simulink model "TP8_gestion_allumage_moteur"  (R2022b)
settings: Solver=VariableStepAuto  StartTime=0.0  StopTime=25  RelTol=1e-3
libraries: simulink x8, fl_lib x7, nesl_utility x4, ee_lib x2
settings Model: Creator=HP  LastModifiedBy=HP

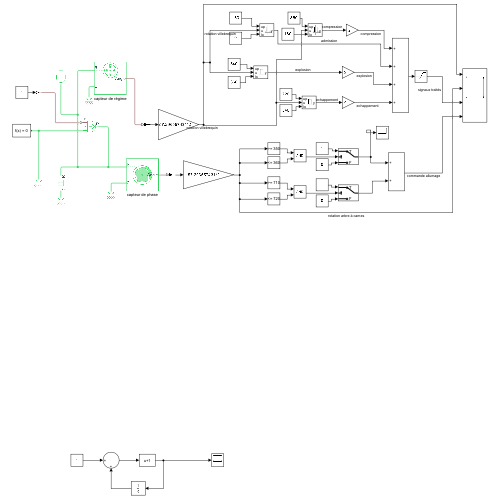
[thumbnail: Simulink's stored preview of the top-level diagram]
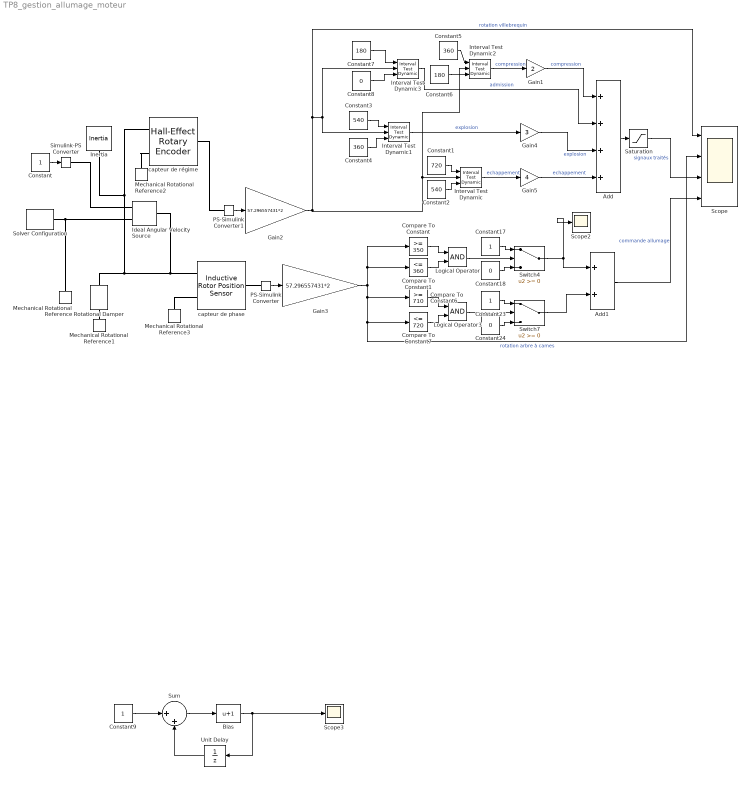
== system TP8_gestion_allumage_moteur ==
  Add : Sum  Inputs=++++
  Add1 : Sum
  Bias : Bias  Bias=1  SaturateOnIntegerOverflow=off
  Compare To Constant : simulink/Logic and Bit Operations/Compare To Constant  relop=>=  const=350  OutDataTypeStr=boolean
  Compare To Constant1 : simulink/Logic and Bit Operations/Compare To Constant  relop=<=  const=360  OutDataTypeStr=boolean
  Compare To Constant6 : simulink/Logic and Bit Operations/Compare To Constant  relop=>=  const=710  OutDataTypeStr=boolean
  Compare To Constant7 : simulink/Logic and Bit Operations/Compare To Constant  relop=<=  const=720  OutDataTypeStr=boolean
  Constant{,9,17,23} (4 alike) : Constant
  Constant1 : Constant  Value=720
  Constant18 : Constant  Value=0
  Constant2 : Constant  Value=540
  Constant24 : Constant  Value=0
  Constant3 : Constant  Value=540
  Constant4 : Constant  Value=360
  Constant5 : Constant  Value=360
  Constant6 : Constant  Value=180
  Constant7 : Constant  Value=180
  Constant8 : Constant  Value=0
  Gain1 : Gain  Gain=2
  Gain2 : Gain  Gain=57.296557431*2
  Gain3 : Gain  Gain=57.296557431*2
  Gain4 : Gain  Gain=3
  Gain5 : Gain  Gain=4
  Ideal Angular Velocity Source : fl_lib/Mechanical/Mechanical Sources/Ideal Angular Velocity Source
  Inertia : fl_lib/Mechanical/Rotational Elements/Inertia  inertia=0.01 kg*m^2  num_ports=foundation.enum.numPorts2.one  w_specify=on  w_priority=None  w=0 rad/s  w_nominal_specify=off  w_nominal_unit=rad/s  w_nominal_value=1  t_specify=off  t_priority=None  t=0 N*m  t_nominal_specify=off  t_nominal_unit=N*m  t_nominal_value=1
  Interval Test Dynamic{,1..3} (4 alike) : simulink/Logic and Bit Operations/Interval Test Dynamic  IntervalClosedRight=on  IntervalClosedLeft=on  OutDataTypeStr=boolean
  Logical Operator : Logic  AllPortsSameDT=off  OutDataTypeStr=boolean
  Logical Operator3 : Logic  AllPortsSameDT=off  OutDataTypeStr=boolean
  Mechanical Rotational Reference{,1..3} (4 alike) : fl_lib/Mechanical/Rotational Elements/Mechanical Rotational Reference
  PS-Simulink Converter : nesl_utility/PS-Simulink Converter  PhysicalDomain=network_engine_domain  SubClassName=ps_output  LeftPortType=input  RightPortType=output  PseudoPeriodic=off  Frequencies=[]  VectorFormat=inherit  Unit=inherit  AffineConversion=off
  PS-Simulink Converter1 : nesl_utility/PS-Simulink Converter  PhysicalDomain=network_engine_domain  SubClassName=ps_output  LeftPortType=input  RightPortType=output  PseudoPeriodic=off  Frequencies=[]  VectorFormat=inherit  Unit=inherit  AffineConversion=off
  Rotational Damper : fl_lib/Mechanical/Rotational Elements/Rotational Damper  D=0.001 N*m*s/rad  w_specify=off  w_priority=None  w=0 rad/s  w_nominal_specify=off  w_nominal_unit=rad/s  w_nominal_value=1  t_specify=off  t_priority=None  t=0 N*m  t_nominal_specify=off  t_nominal_unit=N*m  t_nominal_value=1
  Saturation : Saturate  UpperLimit=4  LowerLimit=1
  Scope : Scope  NumInputPorts=4
  Scope2 : Scope
  Scope3 : Scope
  Simulink-PS Converter : nesl_utility/Simulink-PS Converter  PhysicalDomain=network_engine_domain  SubClassName=ps_input  LeftPortType=input  RightPortType=output  PseudoPeriodic=off  Frequencies=[]  NoiseDistribution=none  NoiseParameters=[]  Unit=1  AffineConversion=off  FilteringAndDerivatives=provide  SimscapeFilterOrder=1  InputFilterTimeConstant=0.001  UdotUserProvided=0
  Solver Configuration : nesl_utility/Solver Configuration  PhysicalDomain=network_engine_domain  SubClassName=solver  LeftPortType=input  RightPortType=generic  Tones=[]  Harmonics=[]  SimulateNoise=off  Profile=off  UseLocalSampling=off  EnableSwitchedLinearOptims=on  FrequencyDomain=off  UseCCode=off  RelTol=0.001  AbsTol=0.001  MinStep=1e-09  ToWorkspace=off  RevertToSquareIcSolve=off  NumHomotopyIterations=100  PhasorMode=off  PhasorModeNumHarmonics=1  ConsistencySolver=NEWTON_XTOL_AFTER_FTOL  IndexReductionMethod=DerivativeReplacement  DoDC=off  ResidualTolerance=1e-09  ConsistencyTolSource=GLOBAL  ConsistencyAbsTol=0.001  ConsistencyRelTol=0.001  ConsistencyTolFactor=0.001  UseLocalSolver=off  LocalSolverChoice=NE_BACKWARD_EULER_ADVANCER  ResolveIndetEquations=on  FunctionEvalNumThread=1  LocalSolverSampleTime=0.001  DoFixedCost=off  MaxNonlinIter=3  MaxModeIter=2  ComputeImpulses=off  ImpulseIterations=2  LinearAlgebra=auto  LinearAlgebraNumThread=0  EquationFormulation=NE_TIME_EF  DelaysMemoryBudget=1024  AutomaticFiltering=on  FilteringTimeConstant=0.001  PartitionStorageMethod=AS_NEEDED  PartitionMemoryBudget=1024  PartitionMethod=ROBUST
  Sum : Sum  Inputs=|++
  Switch4 : Switch  SaturateOnIntegerOverflow=off  InputSameDT=off
  Switch7 : Switch  SaturateOnIntegerOverflow=off  InputSameDT=off
  Unit Delay : UnitDelay  SampleTime=-1  HasFrameUpgradeWarning=on
  capteur de phase : ee_lib/Sensors & Transducers/Inductive Rotor Position Sensor  N=2  Ax=2.5 V  Ay=2.5 V  Vx0=0 V  Vy0=0 V  beta=0 deg  K=0  sensor_output=ee.enum.rotarysensors.output.decoded_ps  theta_specify=off  theta_priority=High  theta=0 deg  theta_nominal_specify=off  theta_nominal_unit=deg  theta_nominal_value=1
      settings: InternalSimscapePortConfiguration="{\"Bottom\":[],\"Left\":[{\"id\":\"R\",\"label\":\"R\",\"type\":\"foundation.mechanical.rotational.rotational\"},{\"id\":\"C\",\"label\":\"C\",\"type\":\"foundation.mechanical.rotational.rotational\"}],\"Right\":[{\"id\":\"A\",\"label\":\"Angle\",\"type\":\"output\"}],\"Top\":[]}"
  capteur de régime : ee_lib/Sensors & Transducers/Hall-Effect Rotary Encoder  Ax=2.5 V  Ay=2.5 V  Vx0=0 V  Vy0=0 V  beta=0 deg  sensor_output=ee.enum.rotarysensors.output.decoded_ps  theta_specify=off  theta_priority=High  theta=0 deg  theta_nominal_specify=off  theta_nominal_unit=deg  theta_nominal_value=1
      settings: InternalSimscapePortConfiguration="{\"Bottom\":[],\"Left\":[{\"id\":\"R\",\"label\":\"R\",\"type\":\"foundation.mechanical.rotational.rotational\"},{\"id\":\"C\",\"label\":\"C\",\"type\":\"foundation.mechanical.rotational.rotational\"}],\"Right\":[{\"id\":\"A\",\"label\":\"Angle\",\"type\":\"output\"}],\"Top\":[]}"
  wires:
  Constant/1 -> Simulink-PS Converter/1
  PS-Simulink Converter1/1 -> Gain2/1
  Constant1/1 -> Interval Test Dynamic/1
  Constant2/1 -> Interval Test Dynamic/3
  Interval Test Dynamic/1 -> Gain5/1  "echappement"
  PS-Simulink Converter/1 -> Gain3/1
  Constant4/1 -> Interval Test Dynamic1/3
  Constant3/1 -> Interval Test Dynamic1/1
  Constant5/1 -> Interval Test Dynamic2/1
  Constant6/1 -> Interval Test Dynamic2/3
  Interval Test Dynamic2/1 -> Gain1/1  "compression"
  Constant8/1 -> Interval Test Dynamic3/3
  Constant7/1 -> Interval Test Dynamic3/1
  Interval Test Dynamic3/1 -> Add/2  "admission"
  Interval Test Dynamic1/1 -> Gain4/1  "explosion"
  Gain1/1 -> Add/1  "compression"
  Gain4/1 -> Add/3  "explosion"
  Gain5/1 -> Add/4  "echappement"
  Add/1 -> Saturation/1
  Saturation/1 -> Scope/3  "signaux traités"
  Gain2/1 -> Interval Test Dynamic2/2, Interval Test Dynamic/2, Interval Test Dynamic1/2, Interval Test Dynamic3/2, Scope/1  "rotation villebrequin"
  Constant9/1 -> Sum/1
  Sum/1 -> Bias/1
  Bias/1 -> Scope3/1, Unit Delay/1
  Unit Delay/1 -> Sum/2
  Logical Operator3/1 -> Switch7/2
  Constant24/1 -> Switch7/3
  Constant17/1 -> Switch4/1
  Add1/1 -> Scope/4  "commande allumage"
  Constant23/1 -> Switch7/1
  Compare To Constant6/1 -> Logical Operator3/1
  Compare To Constant1/1 -> Logical Operator/2
  Switch4/1 -> Scope2/1, Add1/1
  Compare To Constant/1 -> Logical Operator/1
  Switch7/1 -> Add1/2
  Compare To Constant7/1 -> Logical Operator3/2
  Constant18/1 -> Switch4/3
  Logical Operator/1 -> Switch4/2
  Gain3/1 -> Scope/2, Compare To Constant7/1, Compare To Constant6/1, Compare To Constant/1, Compare To Constant1/1  "rotation arbre à cames"
  connections:
  Simulink-PS Converter/RConn1 -- Ideal Angular Velocity Source/RConn1
  Mechanical Rotational Reference/LConn1 -- Solver Configuration/RConn1 -- Ideal Angular Velocity Source/RConn2
  Rotational Damper/RConn1 -- Mechanical Rotational Reference1/LConn1
  capteur de régime/LConn1 -- Inertia/LConn1 -- Rotational Damper/LConn1 -- capteur de phase/LConn1 -- Ideal Angular Velocity Source/LConn1
  PS-Simulink Converter/LConn1 -- capteur de phase/RConn1
  PS-Simulink Converter1/LConn1 -- capteur de régime/RConn1
  capteur de régime/LConn2 -- Mechanical Rotational Reference2/LConn1
  capteur de phase/LConn2 -- Mechanical Rotational Reference3/LConn1
